simulink model "solar_chain_template"  (R2025b)
settings: Solver=FixedStepDiscrete  StartTime=0.0  StopTime=60  FixedStep=p.sim.Ts  RelTol=1e-3
values from neighbouring files (symbols this model uses):
  p = params_sev()    [build_sev.m]    (also in build_solar.m = params_solar(); check_stage1.m; run_solar.m = params_solar())
undefined symbols (not defined in the file or in its folder): Ion, Lithium
libraries: spsGroundLib x3, spsControlledCurrentSourceLib x3, spsCurrentMeasurementLib x2, spsVoltageMeasurementLib x2, spsBatteryLib x1, spsSeriesRLCBranchLib x1, spsPVArrayLib x1, spspowerguiLib x1
settings Model: Creator=jonat  LastModifiedBy=jonat

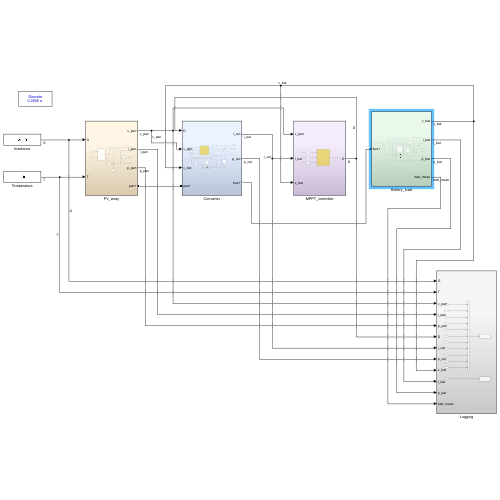
[thumbnail: Simulink's stored preview of the top-level diagram]
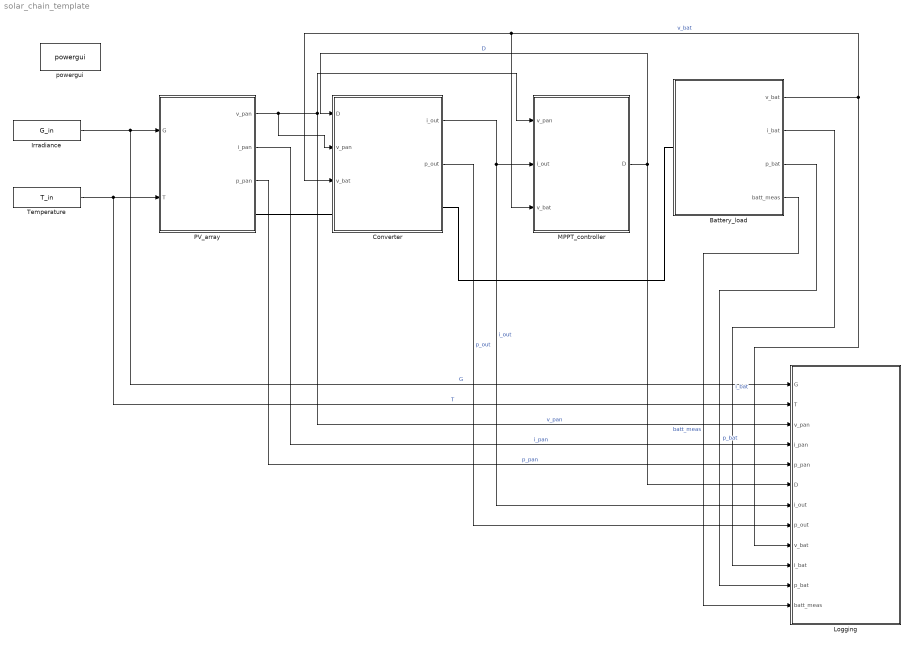
== system solar_chain_template ==
  Battery_load : Subsystem
  Converter : Subsystem
  Irradiance : FromWorkspace  VariableName=G_in  Interpolate=off  OutputAfterFinalValue=Holding final value
  Logging : Subsystem
  MPPT_controller : Subsystem
  PV_array : Subsystem
  Temperature : FromWorkspace  VariableName=T_in  Interpolate=off  OutputAfterFinalValue=Holding final value
  powergui : spspowerguiLib/powergui  Priority=1  SimulationMode=Discrete  SampleTime=p.sim.Ts  frequency=60  Iterations=50  frequencyindice=60  Pbase=100e6  ErrMax=1e-4  UnitsV=kV  UnitsW=MW  buscounter=0  FunctionMessages=off  echomessages=off  EnableUseOfTLC=off  CurrentSourceSwitches=off  DisableSnubberDevices=off  DisableRonSwitches=off  DisableVfSwitches=off  DisplayEquations=off  AutomaticDiscreteSolvers=off  SolverType=Tustin/Backward Euler (TBE)  Interpol=off  ExternalGateDelay=off  methode=off  Ts=100  x0status=blocks  SPID=on  SwTol=0  HookPort=off  NonlinearTolerance=1e-4  nMaxIteration=100  ContinueOnMaxIteration=off  RestoreLinks=warning  ResistiveCurrentMeasurement=off  Frange=[0:2:500]  Ylog=off  Xlog=on  ShowGrid=off  save=off  variable=ZData  structure=0  ZoomFFT=off  StartTime=0.0  cycles=1  DisplayStyle=1  fundamental=60  FreqAxis=off  MaxFrequency=1000  frequencyindicesteady=1  RmsSteady=1  display=off
  wires:
  Irradiance/1 -> PV_array/1(G), Logging/1(G)  "G"
  Temperature/1 -> Logging/2(T), PV_array/2(T)  "T"
  MPPT_controller/1(D) -> Converter/1(D), Logging/6(D)  "D"
  PV_array/1(v_pan) -> Logging/3(v_pan), MPPT_controller/1(v_pan), Converter/2(v_pan)  "v_pan"
  Battery_load/1(v_bat) -> Logging/9(v_bat), MPPT_controller/3(v_bat), Converter/3(v_bat)  "v_bat"
  Converter/1(i_out) -> MPPT_controller/2(i_out), Logging/7(i_out)  "i_out"
  PV_array/2(i_pan) -> Logging/4(i_pan)  "i_pan"
  PV_array/3(p_pan) -> Logging/5(p_pan)  "p_pan"
  Converter/2(p_out) -> Logging/8(p_out)  "p_out"
  Battery_load/2(i_bat) -> Logging/10(i_bat)  "i_bat"
  Battery_load/3(p_bat) -> Logging/11(p_bat)  "p_bat"
  Battery_load/4(batt_meas) -> Logging/12(batt_meas)  "batt_meas"
  connections:
  PV_array/RConn1 -- Converter/LConn1
  Converter/RConn1 -- Battery_load/LConn1

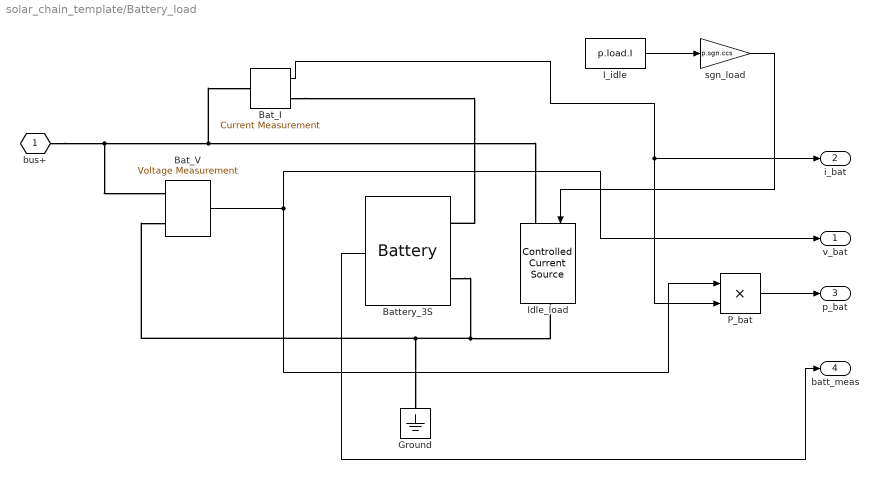
== system solar_chain_template/Battery_load ==
  Bat_I : spsCurrentMeasurementLib/Current Measurement  PhasorSimulation=off  OutputType=Complex  PSBequivalent=0
  Bat_V : spsVoltageMeasurementLib/Voltage Measurement  PhasorSimulation=off  OutputType=Complex  PSBequivalent=0
  Battery_3S : spsBatteryLib/Battery  BatType=Lithium-Ion  NomV=p.batt.Vnom  NomQ=p.batt.Q  SOC=p.batt.SOC0  Batt_Tr=p.batt.Tr  PresetModel=off  MaxQ=p.batt.Q  MinV=p.batt.Vmin  FullV=p.batt.Vfull  Dis_rate=p.batt.Inom  R=p.batt.R  Normal_OP=p.batt.Qnomv  expZone=[p.batt.Vexp p.batt.Qexp]
  Ground : spsGroundLib/Ground  LConnTagsString=a
  I_idle : Constant  Value=p.load.I
  Idle_load : spsControlledCurrentSourceLib/Controlled Current Source  Initialize=off  Source_Type=AC  Amplitude=0  Phase=0  Frequency=0  Measurements=None
  P_bat : Product
  sgn_load : Gain  Gain=p.sgn.ccs
  bus+ : PMIOPort  Side=Left
  v_bat : Outport
  i_bat : Outport  Port=2
  p_bat : Outport  Port=3
  batt_meas : Outport  Port=4
  wires:
  I_idle/1 -> sgn_load/1
  sgn_load/1 -> Idle_load/1
  Bat_V/1 -> P_bat/1, v_bat/1
  Bat_I/1 -> i_bat/1, P_bat/2
  P_bat/1 -> p_bat/1
  Battery_3S/1 -> batt_meas/1
  connections:
  bus+/RConn1 -- Bat_I/LConn1 -- Idle_load/LConn1 -- Bat_V/LConn1
  Bat_I/RConn1 -- Battery_3S/LConn1
  Idle_load/RConn1 -- Ground/LConn1 -- Bat_V/LConn2 -- Battery_3S/LConn2

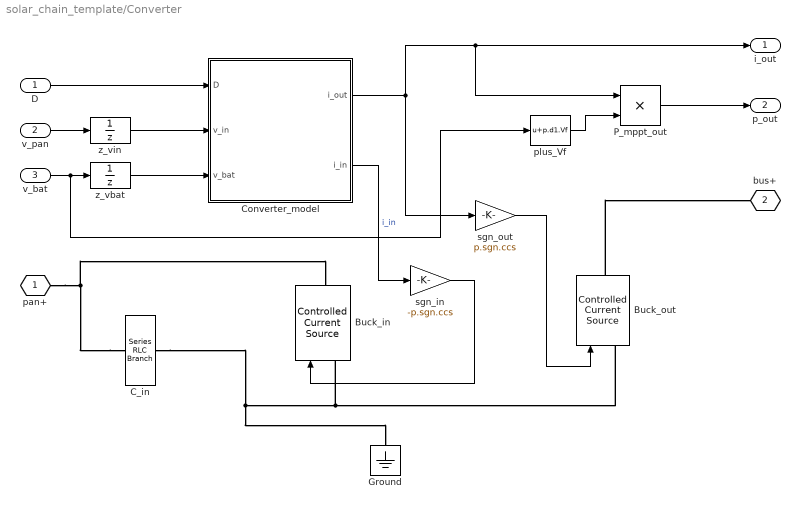
== system solar_chain_template/Converter ==
  D : Inport
  v_pan : Inport  Port=2
  v_bat : Inport  Port=3
  Buck_in : spsControlledCurrentSourceLib/Controlled Current Source  Initialize=off  Source_Type=AC  Amplitude=0  Phase=0  Frequency=0  Measurements=None
  Buck_out : spsControlledCurrentSourceLib/Controlled Current Source  Initialize=off  Source_Type=AC  Amplitude=0  Phase=0  Frequency=0  Measurements=None
  C_in : spsSeriesRLCBranchLib/Series RLC Branch  LConnTagsString=__new0  RConnTagsString=__new0  BranchType=C  Resistance=1  Inductance=1e-3  SetiL0=off  InitialCurrent=0  Capacitance=p.mppt.Cin  Setx0=off  InitialVoltage=0  Measurements=None
  Converter_model : Subsystem
  Ground : spsGroundLib/Ground  LConnTagsString=a
  P_mppt_out : Product
  plus_Vf : Bias  Bias=p.d1.Vf  SaturateOnIntegerOverflow=off
  sgn_in : Gain  Gain=-p.sgn.ccs
  sgn_out : Gain  Gain=p.sgn.ccs
  z_vbat : UnitDelay  InitialCondition=p.batt.Vnom  SampleTime=p.sim.Ts  HasFrameUpgradeWarning=on
  z_vin : UnitDelay  SampleTime=p.sim.Ts  HasFrameUpgradeWarning=on
  pan+ : PMIOPort  Side=Left
  bus+ : PMIOPort  Port=2  Side=Right
  i_out : Outport
  p_out : Outport  Port=2
  wires:
  D/1 -> Converter_model/1(D)
  v_pan/1 -> z_vin/1
  z_vin/1 -> Converter_model/2(v_in)
  v_bat/1 -> plus_Vf/1, z_vbat/1
  z_vbat/1 -> Converter_model/3(v_bat)
  Converter_model/2(i_in) -> sgn_in/1  "i_in"
  sgn_in/1 -> Buck_in/1
  Converter_model/1(i_out) -> P_mppt_out/1, i_out/1, sgn_out/1
  sgn_out/1 -> Buck_out/1
  plus_Vf/1 -> P_mppt_out/2
  P_mppt_out/1 -> p_out/1
  connections:
  C_in/LConn1 -- pan+/RConn1 -- Buck_in/RConn1
  Buck_out/RConn1 -- bus+/RConn1
  Buck_in/LConn1 -- C_in/RConn1 -- Ground/LConn1 -- Buck_out/LConn1

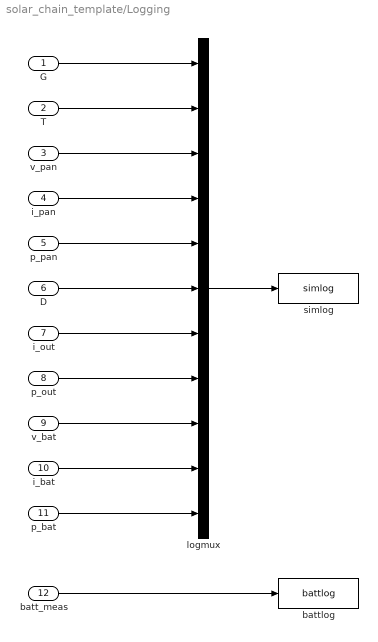
== system solar_chain_template/Logging ==
  G : Inport
  T : Inport  Port=2
  v_pan : Inport  Port=3
  i_pan : Inport  Port=4
  p_pan : Inport  Port=5
  D : Inport  Port=6
  i_out : Inport  Port=7
  p_out : Inport  Port=8
  v_bat : Inport  Port=9
  i_bat : Inport  Port=10
  p_bat : Inport  Port=11
  batt_meas : Inport  Port=12
  battlog : ToWorkspace  VariableName=battlog  SaveFormat=Timeseries  SampleTime=-1
      settings: Decimation=max(1,round(p.sim.Tlog/p.sim.Ts))
  logmux : Mux  Inputs=11
  simlog : ToWorkspace  VariableName=simlog  SaveFormat=Structure With Time  SampleTime=-1
      settings: Decimation=max(1,round(p.sim.Tlog/p.sim.Ts))
  wires:
  G/1 -> logmux/1
  T/1 -> logmux/2
  v_pan/1 -> logmux/3
  i_pan/1 -> logmux/4
  p_pan/1 -> logmux/5
  D/1 -> logmux/6
  i_out/1 -> logmux/7
  p_out/1 -> logmux/8
  v_bat/1 -> logmux/9
  i_bat/1 -> logmux/10
  p_bat/1 -> logmux/11
  logmux/1 -> simlog/1
  batt_meas/1 -> battlog/1

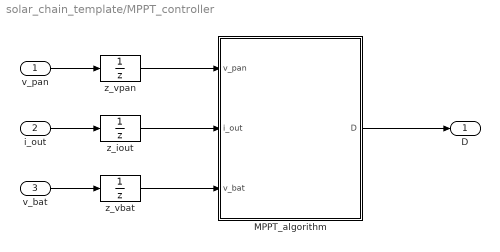
== system solar_chain_template/MPPT_controller ==
  v_pan : Inport
  i_out : Inport  Port=2
  v_bat : Inport  Port=3
  MPPT_algorithm : Subsystem
  z_iout : UnitDelay  SampleTime=p.sim.Ts  HasFrameUpgradeWarning=on
  z_vbat : UnitDelay  InitialCondition=p.batt.Vnom  SampleTime=p.sim.Ts  HasFrameUpgradeWarning=on
  z_vpan : UnitDelay  SampleTime=p.sim.Ts  HasFrameUpgradeWarning=on
  D : Outport
  wires:
  v_pan/1 -> z_vpan/1
  i_out/1 -> z_iout/1
  v_bat/1 -> z_vbat/1
  z_vpan/1 -> MPPT_algorithm/1(v_pan)
  z_iout/1 -> MPPT_algorithm/2(i_out)
  z_vbat/1 -> MPPT_algorithm/3(v_bat)
  MPPT_algorithm/1(D) -> D/1

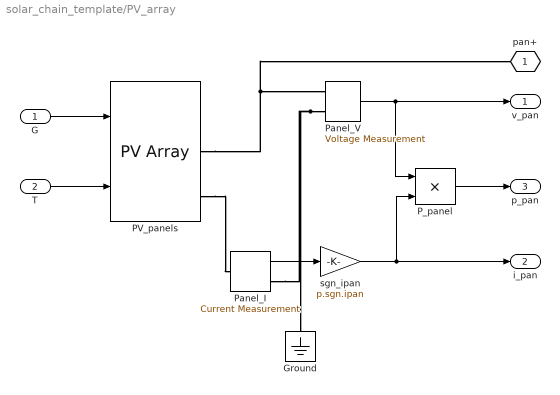
== system solar_chain_template/PV_array ==
  G : Inport
  T : Inport  Port=2
  Ground : spsGroundLib/Ground  LConnTagsString=a
  PV_panels : spsPVArrayLib/PV Array  Npar=1  Nser=2  PlotType=array @ 1000 W/m2 & specified temperatures  S_vec="[ 1000  500  100 ]"  Temp_C_vec="[ 45 25  ]"  ModuleName=User-defined  PlotWhenSelected=off  Pm=7.2  Ncell=18  Voc=11.255  Isc=0.894  Vm=9  Im=0.8  beta_Voc_pc=-0.373  alpha_Isc_pc=0.087  beta_Voc=-0.041981  alpha_Isc=0.00077778  IL=0.89932  I0=4.8298e-11  nI=1.0323  Rsh=178.7086  Rs=1.064  RobustModel=off  RobustCellTemperature=313.3991  BAL=on  Tc=1e-6  Tfilter=5e-5
  P_panel : Product
  Panel_I : spsCurrentMeasurementLib/Current Measurement  PhasorSimulation=off  OutputType=Complex  PSBequivalent=0
  Panel_V : spsVoltageMeasurementLib/Voltage Measurement  PhasorSimulation=off  OutputType=Complex  PSBequivalent=0
  sgn_ipan : Gain  Gain=p.sgn.ipan
  pan+ : PMIOPort  Side=Right
  v_pan : Outport
  i_pan : Outport  Port=2
  p_pan : Outport  Port=3
  wires:
  G/1 -> PV_panels/1
  T/1 -> PV_panels/2
  Panel_I/1 -> sgn_ipan/1
  Panel_V/1 -> P_panel/1, v_pan/1
  sgn_ipan/1 -> i_pan/1, P_panel/2
  P_panel/1 -> p_pan/1
  connections:
  PV_panels/RConn1 -- Panel_V/LConn1 -- pan+/RConn1
  PV_panels/RConn2 -- Panel_I/LConn1
  Panel_V/LConn2 -- Panel_I/RConn1 -- Ground/LConn1

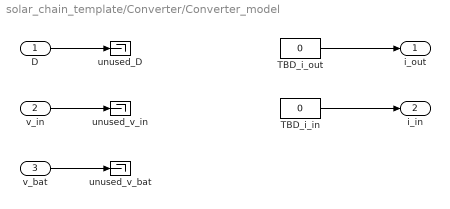
== system solar_chain_template/Converter/Converter_model ==
  D : Inport
  v_in : Inport  Port=2
  v_bat : Inport  Port=3
  TBD_i_in : Constant  Value=0
  TBD_i_out : Constant  Value=0
  unused_D : Terminator
  unused_v_bat : Terminator
  unused_v_in : Terminator
  i_out : Outport
  i_in : Outport  Port=2
  wires:
  D/1 -> unused_D/1
  v_in/1 -> unused_v_in/1
  v_bat/1 -> unused_v_bat/1
  TBD_i_out/1 -> i_out/1
  TBD_i_in/1 -> i_in/1

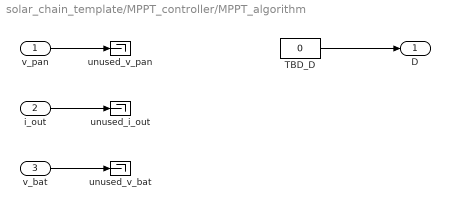
== system solar_chain_template/MPPT_controller/MPPT_algorithm ==
  v_pan : Inport
  i_out : Inport  Port=2
  v_bat : Inport  Port=3
  TBD_D : Constant  Value=0
  unused_i_out : Terminator
  unused_v_bat : Terminator
  unused_v_pan : Terminator
  D : Outport
  wires:
  v_pan/1 -> unused_v_pan/1
  i_out/1 -> unused_i_out/1
  v_bat/1 -> unused_v_bat/1
  TBD_D/1 -> D/1
